simulink model "hunt_hunter_Equation"  (R2024a)
settings: Solver=VariableStepAuto  StartTime=0.0  StopTime=100.0  RelTol=1e-3
settings Model: Creator=Sanagostar  LastModifiedBy=Sanagostar

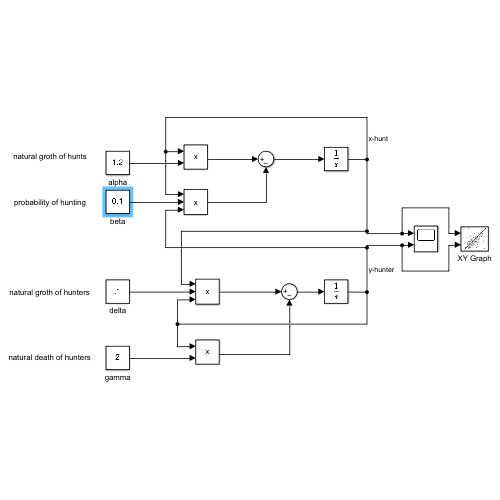
[thumbnail: Simulink's stored preview of the top-level diagram]
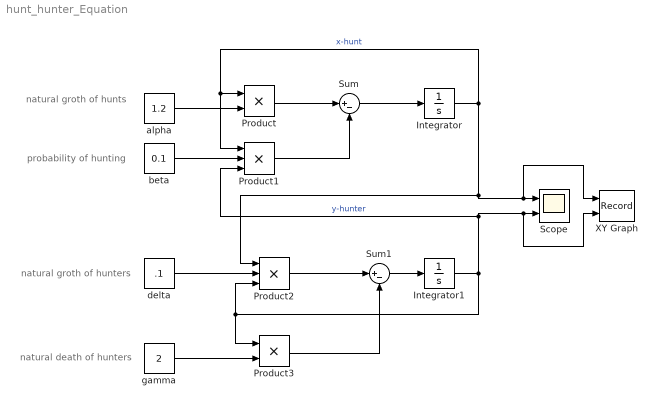
== system hunt_hunter_Equation ==
  note: natural death of hunters
  note: natural groth of hunters
  note: probability of hunting
  note: natural groth of hunts
  Integrator : Integrator  InitialCondition=100
  Integrator1 : Integrator  InitialCondition=20
  Product : Product
  Product1 : Product  Inputs=3
  Product2 : Product  Inputs=3
  Product3 : Product
  Scope : Scope  NumInputPorts=2
  Sum : Sum  Inputs=|+-
  Sum1 : Sum  Inputs=|+-
  XY Graph : Record  FileSettingsInternal="{\"entries\":[{\"content\":{\"excelSettings\":{\"content\":{},\"type\":\"Streamout.ExcelSettings\"}},\"type\":\"Streamout.FileSettingStorage\",\"uuid\":\"\"}],\"packageUris\":[\"http:\\/\\/schema.mathworks.com\\/mf0\\/streamout_blocks\\/R2020a\"],\"version\":\"1.0\"}"  Layout=[1 1]  SignalsInternal="{\"entries\":[{\"content\":{\"signals\":[{\"content\":{\"blockPath\":[],\"dimensions\":[1],\"domain\":\"\",\"lineColor\":\"#a2142f\",\"plots\":[ 1 ],\"port\":1,\"sid\":[\"\"],\"signalID\":1,\"signalName\":\"x-hunt\"},\"type\":\"RecordBlkView.Signal\",\"uuid\":\"\"},{\"content\":{\"blockPath\":[],\"dimensions\":[1],\"domain\":\"\",\"lineColor\":\"#139fff\",\"plots\":[ 1 ],\"port\":2,\"sid\":[\"\"],\"signalID\":2,\"signalName\":\"y-hunter\"},\"type\":\"RecordBlkView.Signal\",\"uuid\":\"\"}]},\"type\":\"RecordBlkView.InputSignals\",\"uuid\":\"\"}],\"packageUris\":[\"http:\\/\\/schema.mathworks.com\\/mf0\\/streamout_blocks\\/R2020a\"],\"version\":\"1.0\"}"  VisualizationBindings="{\"xyplotplugin\":{\"info\":[{\"series\":[{\"bindingParametersList\":[{\"parameter\":\"X-Axis\",\"signalID\":1,\"signalName\":\"x-hunt\"},{\"parameter\":\"Y-Axis\",\"signalID\":2,\"signalName\":\"y-hunter\"}],\"seriesID\":0}],\"subplotID\":1}]}}"  CompatibilityTag=XY
  alpha : Constant  Value=1.2
  beta : Constant  Value=0.1
  delta : Constant  Value=.1
  gamma : Constant  Value=2
  wires:
  alpha/1 -> Product/2
  Product/1 -> Sum/1
  Sum/1 -> Integrator/1
  Integrator/1 -> XY Graph/1, Scope/1, Product2/1, Product1/1, Product/1  "x-hunt"
  beta/1 -> Product1/2
  Integrator1/1 -> XY Graph/2, Scope/2, Product1/3, Product3/1, Product2/3  "y-hunter"
  Product1/1 -> Sum/2
  delta/1 -> Product2/2
  Product2/1 -> Sum1/1
  Product3/1 -> Sum1/2
  gamma/1 -> Product3/2
  Sum1/1 -> Integrator1/1
